simulink model "AFC_FFNN_trainbfg_15_15_15_15_Nor_July_15_RepFast"  (R2021a)
settings: Solver=ode15s  StartTime=0.0  StopTime=T  MaxStep=.01  RelTol=1e-3
undefined symbols (not defined in the file): AF_sensor_tol, fault_time, fuel_inj_tol, kappa_tol, MAF_sensor_tol, patch_sig, pump_tol, safe_patch_sig, sw, tau_ww_tol, x_gain, x_offset, y_gain, y_offset
libraries: neural x66, simulink x3
(part 2 of 3)

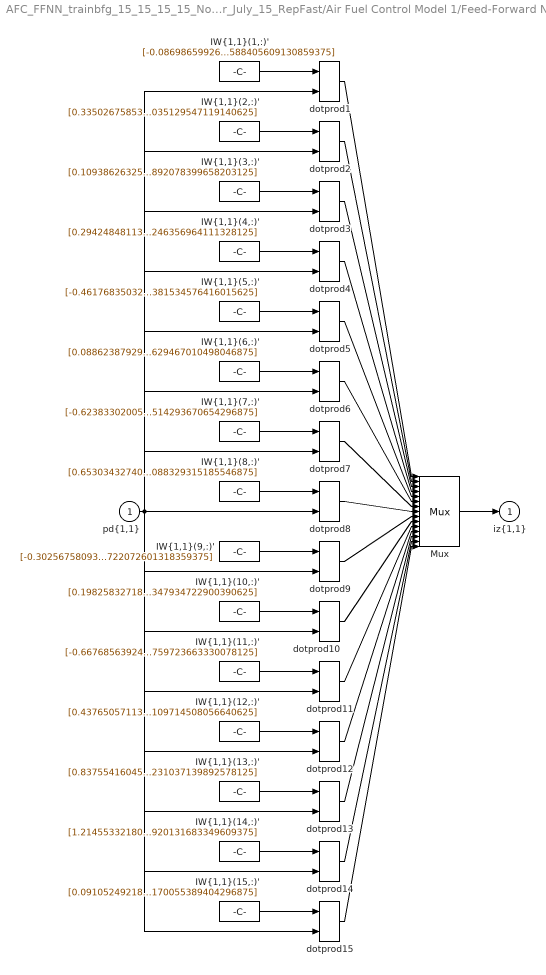
== system AFC_FFNN_trainbfg_15_15_15_15_Nor_July_15_RepFast/Air Fuel Control Model 1/Feed-Forward Neural Network/Layer 1/IW{1,1} ==
  "pd{1,1}" : Inport  PortDimensions=4
      mask Display: e = 0.06;c1 = [120 230 180]/255;c2 = ([120 230 180]+0)/(256+128);c3 = ([120 230 180]+128)/(256+128);patch([0 1 1 0],[0 0 1 1],c1);patch([0 1 1 1-e 1-e 0+e],[0 0 1 1-e 0+e 0+e],c2);patch([0 0 1 1-e 0+e 0+e],[0 1 1 1-e 1-e 0+e],c3);plot([0 1 1 0 0],[0 0 1 1 0]);
  "IW{1,1}(1,:)'" : Constant  Value=[-0.0869865992682361532928325686953030526638031005859375;-0.5106943902266873891448994982056319713592529296875;0.4724684093176680921288834724691696465015411376953125;-0.568692553571918946175856035551987588405609130859375]
      mask Display: e = 0.06;c1 = [120 150 230]/255;c2 = ([120 150 230]+0)/383;c3 = ([120 150 230]+128)/383;patch([0 1 1 0],[0 0 1 1],c1);patch([0 1 1 1-e 1-e 0+e],[0 0 1 1-e 0+e 0+e],c2);patch([0 0 1 1-e 0+e 0+e],[0 1 1 1-e 1-e 0+e],c3);plot([0 1 1 0 0],[0 0 1 1 0]);disp('Weights');
  "IW{1,1}(10,:)'" : Constant  Value=[0.1982583271871785068896087977918796241283416748046875;0.05527160199186720301867126181605271995067596435546875;-0.30839087108283214089254897771752439439296722412109375;-0.8745179996833594149308055420988239347934722900390625]
      mask Display: e = 0.06;c1 = [120 150 230]/255;c2 = ([120 150 230]+0)/383;c3 = ([120 150 230]+128)/383;patch([0 1 1 0],[0 0 1 1],c1);patch([0 1 1 1-e 1-e 0+e],[0 0 1 1-e 0+e 0+e],c2);patch([0 0 1 1-e 0+e 0+e],[0 1 1 1-e 1-e 0+e],c3);plot([0 1 1 0 0],[0 0 1 1 0]);disp('Weights');
  "IW{1,1}(11,:)'" : Constant  Value=[-0.667685639249817608487092002178542315959930419921875;-0.93802145605211040280124734636046923696994781494140625;-0.1853989835261948548872368291995371691882610321044921875;0.56214128127877949214763475538347847759723663330078125]
      mask Display: e = 0.06;c1 = [120 150 230]/255;c2 = ([120 150 230]+0)/383;c3 = ([120 150 230]+128)/383;patch([0 1 1 0],[0 0 1 1],c1);patch([0 1 1 1-e 1-e 0+e],[0 0 1 1-e 0+e 0+e],c2);patch([0 0 1 1-e 0+e 0+e],[0 1 1 1-e 1-e 0+e],c3);plot([0 1 1 0 0],[0 0 1 1 0]);disp('Weights');
  "IW{1,1}(12,:)'" : Constant  Value=[0.43765057113244043573985209150123409926891326904296875;-0.1624415541101225934905727399382158182561397552490234375;0.08024475749677871527776318316682591103017330169677734375;-0.1831281325381338975777367750197299756109714508056640625]
      mask Display: e = 0.06;c1 = [120 150 230]/255;c2 = ([120 150 230]+0)/383;c3 = ([120 150 230]+128)/383;patch([0 1 1 0],[0 0 1 1],c1);patch([0 1 1 1-e 1-e 0+e],[0 0 1 1-e 0+e 0+e],c2);patch([0 0 1 1-e 0+e 0+e],[0 1 1 1-e 1-e 0+e],c3);plot([0 1 1 0 0],[0 0 1 1 0]);disp('Weights');
  "IW{1,1}(13,:)'" : Constant  Value=[0.83755416045026354066038720702636055648326873779296875;0.3011063956881281367117253466858528554439544677734375;1.107514099877665358917511184699833393096923828125;-0.03232339389549805652723790672098402865231037139892578125]
      mask Display: e = 0.06;c1 = [120 150 230]/255;c2 = ([120 150 230]+0)/383;c3 = ([120 150 230]+128)/383;patch([0 1 1 0],[0 0 1 1],c1);patch([0 1 1 1-e 1-e 0+e],[0 0 1 1-e 0+e 0+e],c2);patch([0 0 1 1-e 0+e 0+e],[0 1 1 1-e 1-e 0+e],c3);plot([0 1 1 0 0],[0 0 1 1 0]);disp('Weights');
  "IW{1,1}(14,:)'" : Constant  Value=[1.2145533218092341432026159964152611792087554931640625;0.7268509638130564720626125563285313546657562255859375;0.70797174598533885170326129809836857020854949951171875;0.00154336691632259311555974701235527390963397920131683349609375]
      mask Display: e = 0.06;c1 = [120 150 230]/255;c2 = ([120 150 230]+0)/383;c3 = ([120 150 230]+128)/383;patch([0 1 1 0],[0 0 1 1],c1);patch([0 1 1 1-e 1-e 0+e],[0 0 1 1-e 0+e 0+e],c2);patch([0 0 1 1-e 0+e 0+e],[0 1 1 1-e 1-e 0+e],c3);plot([0 1 1 0 0],[0 0 1 1 0]);disp('Weights');
  "IW{1,1}(15,:)'" : Constant  Value=[0.09105249218804110922231842550900182686746120452880859375;-0.581535088913685438427592089283280074596405029296875;0.93583021448567194067180707861552946269512176513671875;0.08389831398096096737315718883110093884170055389404296875]
      mask Display: e = 0.06;c1 = [120 150 230]/255;c2 = ([120 150 230]+0)/383;c3 = ([120 150 230]+128)/383;patch([0 1 1 0],[0 0 1 1],c1);patch([0 1 1 1-e 1-e 0+e],[0 0 1 1-e 0+e 0+e],c2);patch([0 0 1 1-e 0+e 0+e],[0 1 1 1-e 1-e 0+e],c3);plot([0 1 1 0 0],[0 0 1 1 0]);disp('Weights');
  "IW{1,1}(2,:)'" : Constant  Value=[0.335026758536386193298994840006344020366668701171875;-0.201152411111574114244149313890375196933746337890625;-0.2133049471308530176116846632794477045536041259765625;-0.3964533917460004719401922557153739035129547119140625]
      mask Display: e = 0.06;c1 = [120 150 230]/255;c2 = ([120 150 230]+0)/383;c3 = ([120 150 230]+128)/383;patch([0 1 1 0],[0 0 1 1],c1);patch([0 1 1 1-e 1-e 0+e],[0 0 1 1-e 0+e 0+e],c2);patch([0 0 1 1-e 0+e 0+e],[0 1 1 1-e 1-e 0+e],c3);plot([0 1 1 0 0],[0 0 1 1 0]);disp('Weights');
  "IW{1,1}(3,:)'" : Constant  Value=[0.10938626325194089616843484691344201564788818359375;-0.9510018392496559780369125292054377496242523193359375;0.1800330792084896547322614424047060310840606689453125;-0.680312647265236325466730704647488892078399658203125]
      mask Display: e = 0.06;c1 = [120 150 230]/255;c2 = ([120 150 230]+0)/383;c3 = ([120 150 230]+128)/383;patch([0 1 1 0],[0 0 1 1],c1);patch([0 1 1 1-e 1-e 0+e],[0 0 1 1-e 0+e 0+e],c2);patch([0 0 1 1-e 0+e 0+e],[0 1 1 1-e 1-e 0+e],c3);plot([0 1 1 0 0],[0 0 1 1 0]);disp('Weights');
  "IW{1,1}(4,:)'" : Constant  Value=[0.294248481138897732822812258746125735342502593994140625;1.6834705802136504804167316251550801098346710205078125;1.46690048208046874833598849363625049591064453125;1.00101680340486609566141851246356964111328125]
      mask Display: e = 0.06;c1 = [120 150 230]/255;c2 = ([120 150 230]+0)/383;c3 = ([120 150 230]+128)/383;patch([0 1 1 0],[0 0 1 1],c1);patch([0 1 1 1-e 1-e 0+e],[0 0 1 1-e 0+e 0+e],c2);patch([0 0 1 1-e 0+e 0+e],[0 1 1 1-e 1-e 0+e],c3);plot([0 1 1 0 0],[0 0 1 1 0]);disp('Weights');
  "IW{1,1}(5,:)'" : Constant  Value=[-0.46176835032921481616341452536289580166339874267578125;-0.7029072588150591105460307517205365002155303955078125;0.50750076015753287084208977830712683498859405517578125;-0.53001203028713261833360093078226782381534576416015625]
      mask Display: e = 0.06;c1 = [120 150 230]/255;c2 = ([120 150 230]+0)/383;c3 = ([120 150 230]+128)/383;patch([0 1 1 0],[0 0 1 1],c1);patch([0 1 1 1-e 1-e 0+e],[0 0 1 1-e 0+e 0+e],c2);patch([0 0 1 1-e 0+e 0+e],[0 1 1 1-e 1-e 0+e],c3);plot([0 1 1 0 0],[0 0 1 1 0]);disp('Weights');
  "IW{1,1}(6,:)'" : Constant  Value=[0.08862387929801472663537964535862556658685207366943359375;-0.52399675607354734285792119408142752945423126220703125;0.1790645773388159778249928422155790030956268310546875;-0.434441466979517965096846410233411006629467010498046875]
      mask Display: e = 0.06;c1 = [120 150 230]/255;c2 = ([120 150 230]+0)/383;c3 = ([120 150 230]+128)/383;patch([0 1 1 0],[0 0 1 1],c1);patch([0 1 1 1-e 1-e 0+e],[0 0 1 1-e 0+e 0+e],c2);patch([0 0 1 1-e 0+e 0+e],[0 1 1 1-e 1-e 0+e],c3);plot([0 1 1 0 0],[0 0 1 1 0]);disp('Weights');
  "IW{1,1}(7,:)'" : Constant  Value=[-0.6238330200505395328747226812993176281452178955078125;-0.353668516435942326125996260088868439197540283203125;0.9460228661094201019210458980523981153964996337890625;-0.853042674443184267829565214924514293670654296875]
      mask Display: e = 0.06;c1 = [120 150 230]/255;c2 = ([120 150 230]+0)/383;c3 = ([120 150 230]+128)/383;patch([0 1 1 0],[0 0 1 1],c1);patch([0 1 1 1-e 1-e 0+e],[0 0 1 1-e 0+e 0+e],c2);patch([0 0 1 1-e 0+e 0+e],[0 1 1 1-e 1-e 0+e],c3);plot([0 1 1 0 0],[0 0 1 1 0]);disp('Weights');
  "IW{1,1}(8,:)'" : Constant  Value=[0.65303432740145250789964848081581294536590576171875;0.2217134922507717487150102897430770099163055419921875;-0.29542727021841752588215967989526689052581787109375;-0.629264842459388518136620405130088329315185546875]
      mask Display: e = 0.06;c1 = [120 150 230]/255;c2 = ([120 150 230]+0)/383;c3 = ([120 150 230]+128)/383;patch([0 1 1 0],[0 0 1 1],c1);patch([0 1 1 1-e 1-e 0+e],[0 0 1 1-e 0+e 0+e],c2);patch([0 0 1 1-e 0+e 0+e],[0 1 1 1-e 1-e 0+e],c3);plot([0 1 1 0 0],[0 0 1 1 0]);disp('Weights');
  "IW{1,1}(9,:)'" : Constant  Value=[-0.30256758093461666447865354712121188640594482421875;0.6362068257745299160177410158212296664714813232421875;-0.6001194772566249557854689555824734270572662353515625;-0.1163583691358665017645535044721327722072601318359375]
      mask Display: e = 0.06;c1 = [120 150 230]/255;c2 = ([120 150 230]+0)/383;c3 = ([120 150 230]+128)/383;patch([0 1 1 0],[0 0 1 1],c1);patch([0 1 1 1-e 1-e 0+e],[0 0 1 1-e 0+e 0+e],c2);patch([0 0 1 1-e 0+e 0+e],[0 1 1 1-e 1-e 0+e],c3);plot([0 1 1 0 0],[0 0 1 1 0]);disp('Weights');
  Mux : Mux  Inputs=15
      mask Display: e = 0.06;c1 = [120 150 230]/255;c2 = ([120 150 230]+0)/383;c3 = ([120 150 230]+128)/383;patch([0 1 1 0],[0 0 1 1],c1);patch([0 1 1 1-e 1-e 0+e],[0 0 1 1-e 0+e 0+e],c2);patch([0 0 1 1-e 0+e 0+e],[0 1 1 1-e 1-e 0+e],c3);plot([0 1 1 0 0],[0 0 1 1 0]);disp('Mux');
  dotprod{1..15} (15 alike) : neural/Weight Functions/dotprod
  "iz{1,1}" : Outport
      mask Display: e = 0.06;c1 = [120 230 180]/255;c2 = ([120 230 180]+0)/(256+128);c3 = ([120 230 180]+128)/(256+128);patch([0 1 1 0],[0 0 1 1],c1);patch([0 1 1 1-e 1-e 0+e],[0 0 1 1-e 0+e 0+e],c2);patch([0 0 1 1-e 0+e 0+e],[0 1 1 1-e 1-e 0+e],c3);plot([0 1 1 0 0],[0 0 1 1 0]);
  wires:
  Mux/1 -> "iz{1,1}"/1
  dotprod15/1 -> Mux/15
  "IW{1,1}(15,:)'"/1 -> dotprod15/1
  dotprod14/1 -> Mux/14
  "IW{1,1}(14,:)'"/1 -> dotprod14/1
  dotprod13/1 -> Mux/13
  "IW{1,1}(13,:)'"/1 -> dotprod13/1
  dotprod12/1 -> Mux/12
  "IW{1,1}(12,:)'"/1 -> dotprod12/1
  dotprod11/1 -> Mux/11
  "IW{1,1}(11,:)'"/1 -> dotprod11/1
  dotprod10/1 -> Mux/10
  "IW{1,1}(10,:)'"/1 -> dotprod10/1
  dotprod9/1 -> Mux/9
  "IW{1,1}(9,:)'"/1 -> dotprod9/1
  dotprod8/1 -> Mux/8
  "IW{1,1}(8,:)'"/1 -> dotprod8/1
  dotprod7/1 -> Mux/7
  "IW{1,1}(7,:)'"/1 -> dotprod7/1
  dotprod6/1 -> Mux/6
  "IW{1,1}(6,:)'"/1 -> dotprod6/1
  dotprod5/1 -> Mux/5
  "IW{1,1}(5,:)'"/1 -> dotprod5/1
  dotprod4/1 -> Mux/4
  "IW{1,1}(4,:)'"/1 -> dotprod4/1
  dotprod3/1 -> Mux/3
  "IW{1,1}(3,:)'"/1 -> dotprod3/1
  dotprod2/1 -> Mux/2
  "IW{1,1}(2,:)'"/1 -> dotprod2/1
  dotprod1/1 -> Mux/1
  "pd{1,1}"/1 -> dotprod15/2, dotprod14/2, dotprod13/2, dotprod12/2, dotprod11/2, dotprod10/2, dotprod9/2, dotprod8/2, dotprod7/2, dotprod6/2, dotprod5/2, dotprod4/2, dotprod3/2, dotprod2/2, dotprod1/2
  "IW{1,1}(1,:)'"/1 -> dotprod1/1

== system AFC_FFNN_trainbfg_15_15_15_15_Nor_July_15_RepFast/Air Fuel Control Model 1/Feed-Forward Neural Network/Layer 2/Delays 1 ==
  "p{2}" : Inport  PortDimensions=15
      mask Display: e = 0.06;c1 = [120 230 180]/255;c2 = ([120 230 180]+0)/(256+128);c3 = ([120 230 180]+128)/(256+128);patch([0 1 1 0],[0 0 1 1],c1);patch([0 1 1 1-e 1-e 0+e],[0 0 1 1-e 0+e 0+e],c2);patch([0 0 1 1-e 0+e 0+e],[0 1 1 1-e 1-e 0+e],c3);plot([0 1 1 0 0],[0 0 1 1 0]);
  mux : Mux  Inputs=1
      mask Display: e = 0.06;c1 = [120 150 230]/255;c2 = ([120 150 230]+0)/383;c3 = ([120 150 230]+128)/383;patch([0 1 1 0],[0 0 1 1],c1);patch([0 1 1 1-e 1-e 0+e],[0 0 1 1-e 0+e 0+e],c2);patch([0 0 1 1-e 0+e 0+e],[0 1 1 1-e 1-e 0+e],c3);plot([0 1 1 0 0],[0 0 1 1 0]);disp('Mux')
  "pd{2,1}" : Outport
      mask Display: e = 0.06;c1 = [120 230 180]/255;c2 = ([120 230 180]+0)/(256+128);c3 = ([120 230 180]+128)/(256+128);patch([0 1 1 0],[0 0 1 1],c1);patch([0 1 1 1-e 1-e 0+e],[0 0 1 1-e 0+e 0+e],c2);patch([0 0 1 1-e 0+e 0+e],[0 1 1 1-e 1-e 0+e],c3);plot([0 1 1 0 0],[0 0 1 1 0]);
  wires:
  mux/1 -> "pd{2,1}"/1
  "p{2}"/1 -> mux/1

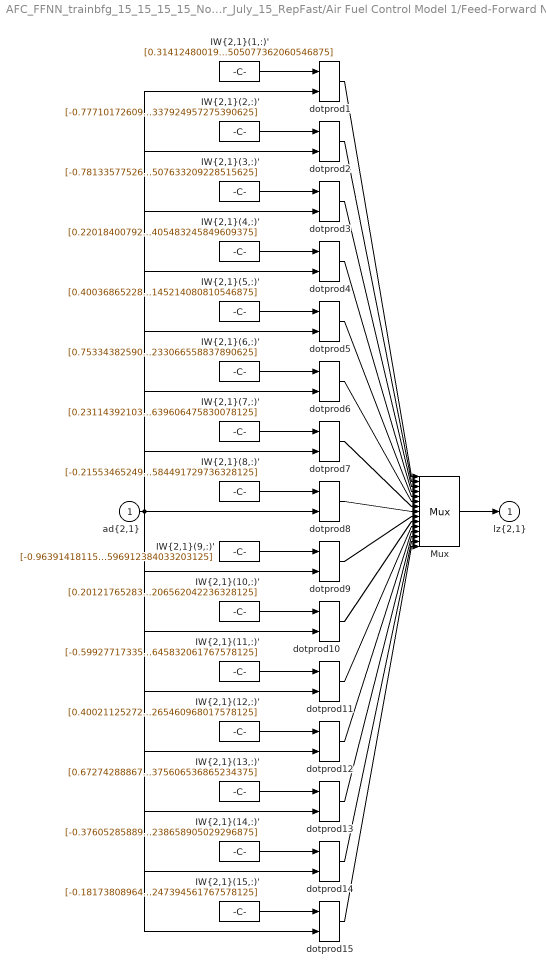
== system AFC_FFNN_trainbfg_15_15_15_15_Nor_July_15_RepFast/Air Fuel Control Model 1/Feed-Forward Neural Network/Layer 2/LW{2,1} ==
  "ad{2,1}" : Inport  PortDimensions=15
      mask Display: e = 0.06;c1 = [120 230 180]/255;c2 = ([120 230 180]+0)/(256+128);c3 = ([120 230 180]+128)/(256+128);patch([0 1 1 0],[0 0 1 1],c1);patch([0 1 1 1-e 1-e 0+e],[0 0 1 1-e 0+e 0+e],c2);patch([0 0 1 1-e 0+e 0+e],[0 1 1 1-e 1-e 0+e],c3);plot([0 1 1 0 0],[0 0 1 1 0]);
  "IW{2,1}(1,:)'" : Constant  Value=[0.314124800191435848972787425736896693706512451171875;0.761219194780894614638100392767228186130523681640625;-0.171753869070582876332764499238692224025726318359375;0.1327757115322516501265681654331274330615997314453125;0.2459442725020564157745184274972416460514068603515625;0.7167434795542131364953775118920020759105682373046875;-0.4743644560107054264364023765665479004383087158203125;0.9964541018726646992575979311368428170680999755859375;-0.3007178641450372058585571721778251230716705322265625;-0.5061911842499977609577399562112987041473388671875;-0.6212526524824333318264280023868195712566375732421875;-0.32664100949461083445157782989554107189178466796875;-0.164745119790139948889873267035000026226043701171875;-0.37571726232811375467690595542080700397491455078125;-0.9219376696445731322882011227193288505077362060546875]
      mask Display: e = 0.06;c1 = [120 150 230]/255;c2 = ([120 150 230]+0)/383;c3 = ([120 150 230]+128)/383;patch([0 1 1 0],[0 0 1 1],c1);patch([0 1 1 1-e 1-e 0+e],[0 0 1 1-e 0+e 0+e],c2);patch([0 0 1 1-e 0+e 0+e],[0 1 1 1-e 1-e 0+e],c3);plot([0 1 1 0 0],[0 0 1 1 0]);disp('weights');
  "IW{2,1}(10,:)'" : Constant  Value=[0.201217652832927473838253717985935509204864501953125;0.7240782555431468647810788752394728362560272216796875;0.8421596785908558313593630373361520469188690185546875;-1.1825149875412674926877798498026095330715179443359375;-0.31519109748938467507883842699811793863773345947265625;-0.795521501318470658503656522952951490879058837890625;0.0713141598183908431707322961301542818546295166015625;-0.0767485023139631294952778262086212635040283203125;-0.1010553699979890307503183066728524863719940185546875;-0.9567843225283756414256686184671707451343536376953125;-0.7217264190297532078233189167804084718227386474609375;0.50100226468314923433666763230576179921627044677734375;0.87766383555333093990924453464685939252376556396484375;0.29681483600678404410899702270398847758769989013671875;0.2310269064815640149834763406033744104206562042236328125]
      mask Display: e = 0.06;c1 = [120 150 230]/255;c2 = ([120 150 230]+0)/383;c3 = ([120 150 230]+128)/383;patch([0 1 1 0],[0 0 1 1],c1);patch([0 1 1 1-e 1-e 0+e],[0 0 1 1-e 0+e 0+e],c2);patch([0 0 1 1-e 0+e 0+e],[0 1 1 1-e 1-e 0+e],c3);plot([0 1 1 0 0],[0 0 1 1 0]);disp('weights');
  "IW{2,1}(11,:)'" : Constant  Value=[-0.5992771733562098912528881555772386491298675537109375;0.1078487493560353893684577997191809117794036865234375;-0.8945967236389289478637465435895137488842010498046875;-0.0500773407099595058156182858510874211788177490234375;0.8870816241124896972536362227401696145534515380859375;0.74014207030404488563135600998066365718841552734375;-0.6866720030229107596397852830705232918262481689453125;0.2726234239649603097177532617934048175811767578125;0.2078428359638626599092958713299594819545745849609375;0.1188907111891503998180041890009306371212005615234375;-0.469008120701347674952330635278485715389251708984375;-0.37068355488443938128284571575932204723358154296875;-0.123525625729133281538452138192951679229736328125;-0.58507783620791808942840361851267516613006591796875;-0.222821272390497870929948476259596645832061767578125]
      mask Display: e = 0.06;c1 = [120 150 230]/255;c2 = ([120 150 230]+0)/383;c3 = ([120 150 230]+128)/383;patch([0 1 1 0],[0 0 1 1],c1);patch([0 1 1 1-e 1-e 0+e],[0 0 1 1-e 0+e 0+e],c2);patch([0 0 1 1-e 0+e 0+e],[0 1 1 1-e 1-e 0+e],c3);plot([0 1 1 0 0],[0 0 1 1 0]);disp('weights');
  "IW{2,1}(12,:)'" : Constant  Value=[0.4002112527225698546118337617372162640094757080078125;0.6440325108893374395080400063307024538516998291015625;0.2318822635474317994663806530297733843326568603515625;-1.2667374338708261571895263841724954545497894287109375;-0.5533384432674870456736471169278956949710845947265625;-0.26613616681114093953652854906977154314517974853515625;0.3727253587085710417881045941612683236598968505859375;0.48813811599891376857840441516600549221038818359375;0.6001589125458657303369136570836417376995086669921875;-0.0802101438462316795874329500293242745101451873779296875;0.65367435221139091883202354438253678381443023681640625;-1.0458216791451082627872892771847546100616455078125;-1.3193113394946169858457096779602579772472381591796875;-0.330369571278571971806314877539989538490772247314453125;0.997369857636166035064206880633719265460968017578125]
      mask Display: e = 0.06;c1 = [120 150 230]/255;c2 = ([120 150 230]+0)/383;c3 = ([120 150 230]+128)/383;patch([0 1 1 0],[0 0 1 1],c1);patch([0 1 1 1-e 1-e 0+e],[0 0 1 1-e 0+e 0+e],c2);patch([0 0 1 1-e 0+e 0+e],[0 1 1 1-e 1-e 0+e],c3);plot([0 1 1 0 0],[0 0 1 1 0]);disp('weights');
  "IW{2,1}(13,:)'" : Constant  Value=[0.67274288867184051099457064992748200893402099609375;0.189393636354295846757622712175361812114715576171875;-0.510549226010743151249471338815055787563323974609375;1.104023685506638319253625013516284525394439697265625;0.8308657357789719366536473899031989276409149169921875;0.367241219801807627920453569458913989365100860595703125;0.8655885705956922748782744747586548328399658203125;-0.0858121130468900705778878545970655977725982666015625;-0.8378375318602981902671444913721643388271331787109375;-0.88685905025613409602414094479172490537166595458984375;0.275859743807580104490995154264965094625949859619140625;0.2062969216335570621367878629826009273529052734375;1.1086902941997625049452835810370743274688720703125;0.442383535765201452161221595815732143819332122802734375;0.95884080775527402717983704860671423375606536865234375]
      mask Display: e = 0.06;c1 = [120 150 230]/255;c2 = ([120 150 230]+0)/383;c3 = ([120 150 230]+128)/383;patch([0 1 1 0],[0 0 1 1],c1);patch([0 1 1 1-e 1-e 0+e],[0 0 1 1-e 0+e 0+e],c2);patch([0 0 1 1-e 0+e 0+e],[0 1 1 1-e 1-e 0+e],c3);plot([0 1 1 0 0],[0 0 1 1 0]);disp('weights');
  "IW{2,1}(14,:)'" : Constant  Value=[-0.3760528588983949038748733073589392006397247314453125;-0.3766582837641696546171488080290146172046661376953125;0.9248846167847240007375830828095786273479461669921875;-0.8676145111114246244454761836095713078975677490234375;0.157385168877649583851763281927560456097126007080078125;-0.4984382819952763998827549585257656872272491455078125;-0.07612045846803727755514046293683350086212158203125;0.1706855767497774678531641256995499134063720703125;0.6769974800018092597753138761618174612522125244140625;0.5403602376259268869063134843599982559680938720703125;-2.3605068409971039500305778346955776214599609375;-0.16106471547288514489792987660621292889118194580078125;-0.369042109842184939960674228132120333611965179443359375;-0.95704290874445641090773051473661325871944427490234375;0.843577088247318140901143124210648238658905029296875]
      mask Display: e = 0.06;c1 = [120 150 230]/255;c2 = ([120 150 230]+0)/383;c3 = ([120 150 230]+128)/383;patch([0 1 1 0],[0 0 1 1],c1);patch([0 1 1 1-e 1-e 0+e],[0 0 1 1-e 0+e 0+e],c2);patch([0 0 1 1-e 0+e 0+e],[0 1 1 1-e 1-e 0+e],c3);plot([0 1 1 0 0],[0 0 1 1 0]);disp('weights');
  "IW{2,1}(15,:)'" : Constant  Value=[-0.1817380896437239545804231966030783951282501220703125;-0.819076525749918626928547382703982293605804443359375;-0.703422130964734382274627932929433882236480712890625;-0.94939269002778214900928333008778281509876251220703125;-0.896269677871021741566437412984669208526611328125;-0.3356003910290790148707174012088216841220855712890625;-0.2214840900786894106744284727028571069240570068359375;-0.4191414392946388733918183788773603737354278564453125;-0.2687179919619584467227468849159777164459228515625;0.98276969821900905799338943324983119964599609375;-0.0363505221006390488724946408183313906192779541015625;-0.55328677456039410120780530633055604994297027587890625;0.89155338038898801489295919964206404983997344970703125;-0.11752903231500504144246832538556191138923168182373046875;-0.79833567739331734447461030867998488247394561767578125]
      mask Display: e = 0.06;c1 = [120 150 230]/255;c2 = ([120 150 230]+0)/383;c3 = ([120 150 230]+128)/383;patch([0 1 1 0],[0 0 1 1],c1);patch([0 1 1 1-e 1-e 0+e],[0 0 1 1-e 0+e 0+e],c2);patch([0 0 1 1-e 0+e 0+e],[0 1 1 1-e 1-e 0+e],c3);plot([0 1 1 0 0],[0 0 1 1 0]);disp('weights');
  "IW{2,1}(2,:)'" : Constant  Value=[-0.7771017260971981865935731548233889043331146240234375;-0.989689411673975616423604151350446045398712158203125;0.85939642766992552225246981834061443805694580078125;-0.61030381879570694270142894310993142426013946533203125;0.30497898667072576017744722776114940643310546875;0.092222522227818071183236270371708087623119354248046875;-0.005466530920209766719608523999340832233428955078125;0.8236928328595840564929631000268273055553436279296875;0.0456944657569839929323052274412475526332855224609375;0.8261448944639935287881371550611220300197601318359375;0.429014213658457210787133817575522698462009429931640625;-0.32131717688586680647944149313843809068202972412109375;-0.52240941017245867694640537592931650578975677490234375;0.29152713968148391554535692193894647061824798583984375;0.494308555574343666538794650477939285337924957275390625]
      mask Display: e = 0.06;c1 = [120 150 230]/255;c2 = ([120 150 230]+0)/383;c3 = ([120 150 230]+128)/383;patch([0 1 1 0],[0 0 1 1],c1);patch([0 1 1 1-e 1-e 0+e],[0 0 1 1-e 0+e 0+e],c2);patch([0 0 1 1-e 0+e 0+e],[0 1 1 1-e 1-e 0+e],c3);plot([0 1 1 0 0],[0 0 1 1 0]);disp('weights');
  "IW{2,1}(3,:)'" : Constant  Value=[-0.7813357752653991017410817221389152109622955322265625;0.2884373573340142105081440604408271610736846923828125;-0.1790504980917517752203593772719614207744598388671875;-0.62459444844897393789295847454923205077648162841796875;0.9792166972620892639866951867588795721530914306640625;-0.05772109104215349117961153524447581730782985687255859375;-0.0859133263877100983307855130988173186779022216796875;-0.903421362694661223002867700415663421154022216796875;-0.3519069100123857207762512189219705760478973388671875;0.68567142254128310430161263866466470062732696533203125;0.427114206938296436799618049917626194655895233154296875;-0.1887415273689747596819188402150757610797882080078125;0.08611314277500585478986039333904045633971691131591796875;0.9918392466822412156801647142856381833553314208984375;-0.8345158850484593049401382813812233507633209228515625]
      mask Display: e = 0.06;c1 = [120 150 230]/255;c2 = ([120 150 230]+0)/383;c3 = ([120 150 230]+128)/383;patch([0 1 1 0],[0 0 1 1],c1);patch([0 1 1 1-e 1-e 0+e],[0 0 1 1-e 0+e 0+e],c2);patch([0 0 1 1-e 0+e 0+e],[0 1 1 1-e 1-e 0+e],c3);plot([0 1 1 0 0],[0 0 1 1 0]);disp('weights');
  "IW{2,1}(4,:)'" : Constant  Value=[0.22018400792110437436122083454392850399017333984375;0.6991144072415418353472205126308836042881011962890625;0.3099402980647762984034443434211425483226776123046875;0.061498952364746749255086655239210813306272029876708984375;0.439963017584670768034271759461262263357639312744140625;0.53700087765160320341095712137757800519466400146484375;-0.9259617635520160927597999034333042800426483154296875;0.6153389276731864310221453706617467105388641357421875;-0.4045481598141231760479286094778217375278472900390625;0.70229649611518774054985669863526709377765655517578125;-1.0632415478873624703481937103788368403911590576171875;1.037732974579840483642101389705203473567962646484375;-0.56732075540575477301530327167711220681667327880859375;0.03649661653649223513884436442822334356606006622314453125;0.6470024656570847465530960107571445405483245849609375]
      mask Display: e = 0.06;c1 = [120 150 230]/255;c2 = ([120 150 230]+0)/383;c3 = ([120 150 230]+128)/383;patch([0 1 1 0],[0 0 1 1],c1);patch([0 1 1 1-e 1-e 0+e],[0 0 1 1-e 0+e 0+e],c2);patch([0 0 1 1-e 0+e 0+e],[0 1 1 1-e 1-e 0+e],c3);plot([0 1 1 0 0],[0 0 1 1 0]);disp('weights');
  "IW{2,1}(5,:)'" : Constant  Value=[0.4003686522850926632344226163695566356182098388671875;0.7154922757569484037531992726144380867481231689453125;-0.55451457198497333678233189857564866542816162109375;-0.701016426748160892401529054041020572185516357421875;0.2719693029116949656298629633965902030467987060546875;0.3452701580345747256473032393842004239559173583984375;-0.9904793588654232650014819228090345859527587890625;0.421753225196830339172038293327204883098602294921875;-0.6134849306530993917618843624950386583805084228515625;0.6205332793438713689937458184431307017803192138671875;-0.2900360464848421582217952163773588836193084716796875;-0.8601594396824143728963463217951357364654541015625;-0.7387104842103118240714820785797201097011566162109375;-0.64540323855050463208726796437986195087432861328125;-0.2133330335187888504577813364448957145214080810546875]
      mask Display: e = 0.06;c1 = [120 150 230]/255;c2 = ([120 150 230]+0)/383;c3 = ([120 150 230]+128)/383;patch([0 1 1 0],[0 0 1 1],c1);patch([0 1 1 1-e 1-e 0+e],[0 0 1 1-e 0+e 0+e],c2);patch([0 0 1 1-e 0+e 0+e],[0 1 1 1-e 1-e 0+e],c3);plot([0 1 1 0 0],[0 0 1 1 0]);disp('weights');
  "IW{2,1}(6,:)'" : Constant  Value=[0.7533438259077460674717485744622536003589630126953125;-0.1622850437559437697387920707114972174167633056640625;-0.2221844078714447778821750034694559872150421142578125;0.54429151285718668784596729892655275762081146240234375;1.00787934291988801049910762230865657329559326171875;0.3163128591791328769744495730265043675899505615234375;0.2893143771285426879558144719339907169342041015625;0.9802256885177147438525935285724699497222900390625;-0.3613982857657287439678839291445910930633544921875;-0.90323576071038391699374869858729653060436248779296875;1.52266978362477178876588368439115583896636962890625;0.414545013788929994635878983899601735174655914306640625;-0.25805726547611007593019394334987737238407135009765625;0.79414819953845261490954499095096252858638763427734375;0.465672824324343537227832712233066558837890625]
      mask Display: e = 0.06;c1 = [120 150 230]/255;c2 = ([120 150 230]+0)/383;c3 = ([120 150 230]+128)/383;patch([0 1 1 0],[0 0 1 1],c1);patch([0 1 1 1-e 1-e 0+e],[0 0 1 1-e 0+e 0+e],c2);patch([0 0 1 1-e 0+e 0+e],[0 1 1 1-e 1-e 0+e],c3);plot([0 1 1 0 0],[0 0 1 1 0]);disp('weights');
  "IW{2,1}(7,:)'" : Constant  Value=[0.23114392103916969745114329271018505096435546875;0.9635763073263967637416271827532909810543060302734375;-0.1671208207308916282585187218501232564449310302734375;0.06329895739177394953234312424683594144880771636962890625;-0.378452929134685034373575263089151121675968170166015625;0.11958422424242327875010261095667374320328235626220703125;-0.607419333399665362094310694374144077301025390625;0.0111096917961808205888019074336625635623931884765625;-0.8105754243397400582438194760470651090145111083984375;0.318929817605345056197307940237806178629398345947265625;-0.7900852178016195548337918808101676404476165771484375;-0.21373528018232745839810604593367315828800201416015625;-0.5969408965863836069587478050380013883113861083984375;-0.90852813610887828144058175894315354526042938232421875;-0.287242937260107134012088181407307274639606475830078125]
      mask Display: e = 0.06;c1 = [120 150 230]/255;c2 = ([120 150 230]+0)/383;c3 = ([120 150 230]+128)/383;patch([0 1 1 0],[0 0 1 1],c1);patch([0 1 1 1-e 1-e 0+e],[0 0 1 1-e 0+e 0+e],c2);patch([0 0 1 1-e 0+e 0+e],[0 1 1 1-e 1-e 0+e],c3);plot([0 1 1 0 0],[0 0 1 1 0]);disp('weights');
  "IW{2,1}(8,:)'" : Constant  Value=[-0.2155346524932839624710823045461438596248626708984375;0.890530830596826472600469060125760734081268310546875;-0.9467920414380841531709620539913885295391082763671875;-0.434011281189908115774045427315286360681056976318359375;0.26579035938519302018079315530485473573207855224609375;0.2172980620921392269639937921965611167252063751220703125;0.292716250101574093633871598285622894763946533203125;0.1305612562825471112404329687706194818019866943359375;-0.871055828832263845384886735701002180576324462890625;-0.17721316472024450927591487925383262336254119873046875;-0.71934773715706235019951009235228411853313446044921875;0.25931984951627884417035829756059683859348297119140625;0.21468822963550027171919509783037938177585601806640625;0.16340570924226149873703661796753294765949249267578125;-0.81406715037500021470151523317326791584491729736328125]
      mask Display: e = 0.06;c1 = [120 150 230]/255;c2 = ([120 150 230]+0)/383;c3 = ([120 150 230]+128)/383;patch([0 1 1 0],[0 0 1 1],c1);patch([0 1 1 1-e 1-e 0+e],[0 0 1 1-e 0+e 0+e],c2);patch([0 0 1 1-e 0+e 0+e],[0 1 1 1-e 1-e 0+e],c3);plot([0 1 1 0 0],[0 0 1 1 0]);disp('weights');
  "IW{2,1}(9,:)'" : Constant  Value=[-0.96391418115658300536097158328630030155181884765625;0.510168063185229225808825503918342292308807373046875;0.312107034951037309866705982130952179431915283203125;0.33415533498262950384827263405895791947841644287109375;0.159088574682244077163062456747866235673427581787109375;0.303936777339137431663829147510114125907421112060546875;-0.06134999454679768149389929021708667278289794921875;-0.769981108969951311138402161304838955402374267578125;-0.5287401885702369686015344996121712028980255126953125;-0.0309998749507064234876008157471005688421428203582763671875;0.18321056239390876019257348161772824823856353759765625;0.0783758268001817637316008813286316581070423126220703125;0.1645435635146068609202529842150397598743438720703125;-1.1439631090601272145335087770945392549037933349609375;0.74931802165753680355919641442596912384033203125]
      mask Display: e = 0.06;c1 = [120 150 230]/255;c2 = ([120 150 230]+0)/383;c3 = ([120 150 230]+128)/383;patch([0 1 1 0],[0 0 1 1],c1);patch([0 1 1 1-e 1-e 0+e],[0 0 1 1-e 0+e 0+e],c2);patch([0 0 1 1-e 0+e 0+e],[0 1 1 1-e 1-e 0+e],c3);plot([0 1 1 0 0],[0 0 1 1 0]);disp('weights');
  Mux : Mux  Inputs=15
      mask Display: e = 0.06;c1 = [120 150 230]/255;c2 = ([120 150 230]+0)/383;c3 = ([120 150 230]+128)/383;patch([0 1 1 0],[0 0 1 1],c1);patch([0 1 1 1-e 1-e 0+e],[0 0 1 1-e 0+e 0+e],c2);patch([0 0 1 1-e 0+e 0+e],[0 1 1 1-e 1-e 0+e],c3);plot([0 1 1 0 0],[0 0 1 1 0]);disp('Mux');
  dotprod{1..15} (15 alike) : neural/Weight Functions/dotprod
  "lz{2,1}" : Outport
      mask Display: e = 0.06;c1 = [120 230 180]/255;c2 = ([120 230 180]+0)/(256+128);c3 = ([120 230 180]+128)/(256+128);patch([0 1 1 0],[0 0 1 1],c1);patch([0 1 1 1-e 1-e 0+e],[0 0 1 1-e 0+e 0+e],c2);patch([0 0 1 1-e 0+e 0+e],[0 1 1 1-e 1-e 0+e],c3);plot([0 1 1 0 0],[0 0 1 1 0]);
  wires:
  Mux/1 -> "lz{2,1}"/1
  dotprod15/1 -> Mux/15
  "IW{2,1}(15,:)'"/1 -> dotprod15/1
  dotprod14/1 -> Mux/14
  "IW{2,1}(14,:)'"/1 -> dotprod14/1
  dotprod13/1 -> Mux/13
  "IW{2,1}(13,:)'"/1 -> dotprod13/1
  dotprod12/1 -> Mux/12
  "IW{2,1}(12,:)'"/1 -> dotprod12/1
  dotprod11/1 -> Mux/11
  "IW{2,1}(11,:)'"/1 -> dotprod11/1
  dotprod10/1 -> Mux/10
  "IW{2,1}(10,:)'"/1 -> dotprod10/1
  dotprod9/1 -> Mux/9
  "IW{2,1}(9,:)'"/1 -> dotprod9/1
  dotprod8/1 -> Mux/8
  "IW{2,1}(8,:)'"/1 -> dotprod8/1
  dotprod7/1 -> Mux/7
  "IW{2,1}(7,:)'"/1 -> dotprod7/1
  dotprod6/1 -> Mux/6
  "IW{2,1}(6,:)'"/1 -> dotprod6/1
  dotprod5/1 -> Mux/5
  "IW{2,1}(5,:)'"/1 -> dotprod5/1
  dotprod4/1 -> Mux/4
  "IW{2,1}(4,:)'"/1 -> dotprod4/1
  dotprod3/1 -> Mux/3
  "IW{2,1}(3,:)'"/1 -> dotprod3/1
  dotprod2/1 -> Mux/2
  "IW{2,1}(2,:)'"/1 -> dotprod2/1
  dotprod1/1 -> Mux/1
  "ad{2,1}"/1 -> dotprod15/2, dotprod14/2, dotprod13/2, dotprod12/2, dotprod11/2, dotprod10/2, dotprod9/2, dotprod8/2, dotprod7/2, dotprod6/2, dotprod5/2, dotprod4/2, dotprod3/2, dotprod2/2, dotprod1/2
  "IW{2,1}(1,:)'"/1 -> dotprod1/1

== system AFC_FFNN_trainbfg_15_15_15_15_Nor_July_15_RepFast/Air Fuel Control Model 1/Feed-Forward Neural Network/Layer 3/Delays 1 ==
  "p{3}" : Inport  PortDimensions=15
      mask Display: e = 0.06;c1 = [120 230 180]/255;c2 = ([120 230 180]+0)/(256+128);c3 = ([120 230 180]+128)/(256+128);patch([0 1 1 0],[0 0 1 1],c1);patch([0 1 1 1-e 1-e 0+e],[0 0 1 1-e 0+e 0+e],c2);patch([0 0 1 1-e 0+e 0+e],[0 1 1 1-e 1-e 0+e],c3);plot([0 1 1 0 0],[0 0 1 1 0]);
  mux : Mux  Inputs=1
      mask Display: e = 0.06;c1 = [120 150 230]/255;c2 = ([120 150 230]+0)/383;c3 = ([120 150 230]+128)/383;patch([0 1 1 0],[0 0 1 1],c1);patch([0 1 1 1-e 1-e 0+e],[0 0 1 1-e 0+e 0+e],c2);patch([0 0 1 1-e 0+e 0+e],[0 1 1 1-e 1-e 0+e],c3);plot([0 1 1 0 0],[0 0 1 1 0]);disp('Mux')
  "pd{3,2}" : Outport
      mask Display: e = 0.06;c1 = [120 230 180]/255;c2 = ([120 230 180]+0)/(256+128);c3 = ([120 230 180]+128)/(256+128);patch([0 1 1 0],[0 0 1 1],c1);patch([0 1 1 1-e 1-e 0+e],[0 0 1 1-e 0+e 0+e],c2);patch([0 0 1 1-e 0+e 0+e],[0 1 1 1-e 1-e 0+e],c3);plot([0 1 1 0 0],[0 0 1 1 0]);
  wires:
  mux/1 -> "pd{3,2}"/1
  "p{3}"/1 -> mux/1
